simulink model "PI_controller"  (R2024b)
settings: Solver=FixedStepDiscrete  StartTime=0.0  StopTime=inf  FixedStep=0.02  RelTol=1e-3
undefined symbols (not defined in the file): brake, steering, throttle
libraries: ros2lib x5, slpidlib x1
settings Model: Creator=haavi  LastModifiedBy=haavi
settings OptimizationCC: DefaultParameterBehavior=Inlined  EnhancedBackFolding=on  PassReuseOutputArgsAs=Individual arguments  ZeroExternalMemoryAtStartup=off  ZeroInternalMemoryAtStartup=off  MaxStackSize=64  OptimizeBlockOrder=speed  DifferentSizesBufferReuse=on  EfficientTunableParamExpr=on
settings DebuggingCC: ParameterTunabilityLossMsg=error
settings SFSimCC: MATLABDynamicMemAlloc=off
settings RTWCC: Description=Embedded Coder  SystemTargetFile=ert.tlc  HardwareBoard=Robot Operating System 2 (ROS 2)  TLCOptions="-aInlineSetEventsForThisBaseRateFcn=TLC_FALSE -aSuppressMultiTaskScheduler=TLC_FALSE  -aRateBasedStepFcn=0"  TemplateMakefile=ert_default_tmf  Toolchain=Colcon Tools  TargetLang=C++
settings CodeAppCC: ForceParamTrailComments=on  IgnoreCustomStorageClasses=off  OperatorAnnotations=on  SimulinkDataObjDesc=on  SFDataObjDesc=on  InsertBlockDesc=on
settings ERTTargetCC: CodeInterfacePackaging=C++ class  SupportContinuousTime=on  RootIOFormat=Structure reference

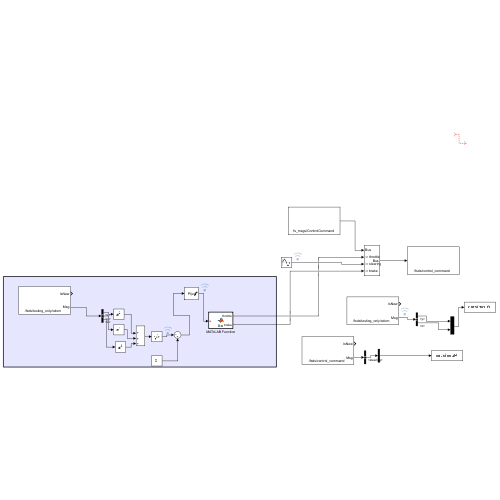
[thumbnail: Simulink's stored preview of the top-level diagram]
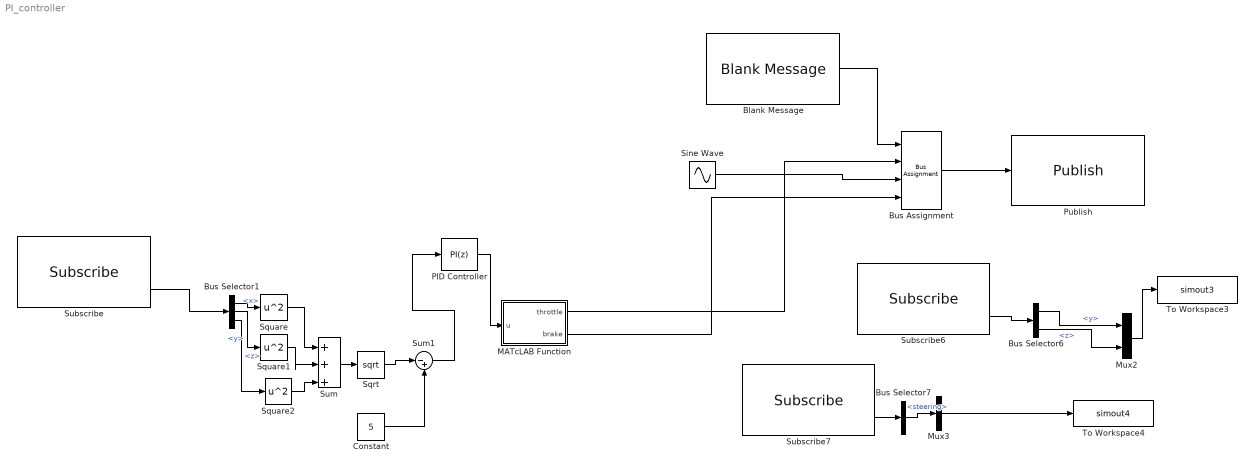
== system PI_controller ==
  Blank Message : ros2lib/Blank Message  messageClass=Message  entityType=fs_msgs/ControlCommand  messageType=fs_msgs/ControlCommand  SampleTime=0.02
  Bus Assignment : BusAssignment  AssignedSignals=throttle,steering,brake
  Bus Selector1 : BusSelector  OutputSignals=twist.twist.linear.x,twist.twist.linear.y,twist.twist.linear.z
  Bus Selector6 : BusSelector  OutputSignals=twist.twist.linear.y,twist.twist.angular.z
  Bus Selector7 : BusSelector  OutputSignals=steering
  Constant : Constant  Value=5
  MATcLAB Function : MATLAB Function  TreatAsAtomicUnit=on
  Mux2 : Mux  Inputs=2
  Mux3 : Mux  Inputs=1
  PID Controller : slpidlib/PID Controller  Controller=PI  Form=Parallel  TimeDomain=Discrete-time  UseExternalTs=off  SampleTime=0.02  IntegratorMethod=Forward Euler  FilterMethod=Forward Euler  ControllerParametersSource=internal  P=0.04  I=0.003  UseKiTs=off  D=0.0003  UseExternalDerivativeSource=off  N=100  UseFilter=off  TunerSelectOption=Transfer Function Based (PID Tuner App)  InitialConditionSource=internal  InitialConditionForIntegrator=0  InitialConditionForFilter=0  DifferentiatorICPrevScaledInput=0  ExternalReset=none  TrackingMode=off  Kt=1  LimitOutput=on  SatLimitsSource=internal  UpperSaturationLimit=1  LowerSaturationLimit=-1  LinearizeAsGain=off  AntiWindupMode=back-calculation  Kb=1  LimitIntegrator=off  UpperIntegratorSaturationLimit=0  LowerIntegratorSaturationLimit=1  POutMin=[]  POutMax=[]  IOutMin=[]  IOutMax=[]  DOutMin=[]  DOutMax=[]  NOutMin=[]  NOutMax=[]  SumOutMin=[]  SumOutMax=[]  SaturationOutMin=[]  SaturationOutMax=[]  PParamMin=[]  PParamMax=[]  IParamMin=[]  IParamMax=[]  DParamMin=[]  DParamMax=[]  NParamMin=[]  NParamMax=[]  KbParamMin=[]  KbParamMax=[]  KtParamMin=[]  KtParamMax=[]  KbOutMin=[]  KbOutMax=[]  KtOutMin=[]  KtOutMax=[]  IntegratorOutMin=[]  IntegratorOutMax=[]  FilterOutMin=[]  FilterOutMax=[]  SumI1OutMin=[]  SumI1OutMax=[]  SumI2OutMin=[]  SumI2OutMax=[]  SumI3OutMin=[]  SumI3OutMax=[]  SumI4OutMin=[]  SumI4OutMax=[]  SumDOutMin=[]  SumDOutMax=[]  DifferentiatorOutMin=[]  DifferentiatorOutMax=[]  FilterDiffOutCoefMin=[]  FilterDiffOutCoefMax=[]  ReciprocalOutMin=[]  ReciprocalOutMax=[]  SumDenOutMin=[]  SumDenOutMax=[]  SumNumOutMin=[]  SumNumOutMax=[]  DivideOutMin=[]  DivideOutMax=[]  UdiffTsProdOutMin=[]  UdiffTsProdOutMax=[]  NTsProdOutMin=[]  NTsProdOutMax=[]  UintegralTsProdOutMin=[]  UintegralTsProdOutMax=[]  UngainTsProdOutMin=[]  UngainTsProdOutMax=[]  ClampingZeroOutDataTypeStr=Inherit: Inherit via back propagation  ClampingZeroOutMin=[]  ClampingZeroOutMax=[]  FilterDenConstantOutDataTypeStr=Inherit: Inherit via back propagation  FilterDenConstantOutMin=[]  FilterDenConstantOutMax=[]  PCopyOutDataTypeStr=Inherit: Inherit via back propagation  PCopyOutMin=[]  PCopyOutMax=[]  NCopyOutDataTypeStr=Inherit: Inherit via back propagation  NCopyOutMin=[]  NCopyOutMax=[]  IntegratorContinuousStateAttributes=''  IntegratorStateMustResolveToSignalObject=off  IntegratorRTWStateStorageClass=Auto  FilterContinuousStateAttributes=''  FilterStateMustResolveToSignalObject=off  FilterRTWStateStorageClass=Auto  ParallelPVariant=InternalParameters  IdealPVariant=Disabled  IVariant=InternalParameters  DVariant=Disabled  IntegratorVariant=Discrete  SatVariant=Enabled  AWVariant=BackCalculation  PCopyVariant=Disabled  TRVariant=Disabled  FdbkBlocksVariant=Forward  IdealPFdbkVariant=Disabled  SatFdbkVariant=Disabled  DerivativeFilterVariant=Disabled  NVariant=Disabled  NCopyVariant=Disabled_SignalSpec  FilterICVariant=Disabled  IntegratorICVariant=InternalICs  ExternalResetVariant=Disabled  TRSumVariant=Passthrough  SumFdbkVariant=Disabled  SumVariant=Sum_PI  TsampFilterVariant=InternalTs  TsampNgainVariant=Passthrough  TsampIntegralVariant=Disabled_SignalSpec  ExternalSaturationOutDataTypeStr=Inherit: Same as second input  DerivativeSourceVariant=Disabled  PreIntVariant=InternalPreInt
  Publish : ros2lib/Publish  topicSource=Select from ROS network  topic=/fsds/control_command  messageType=fs_msgs/ControlCommand  QOSHistory=Keep last  QOSDepth=1  QOSReliability=Reliable  QOSDurability=Volatile  QOSDeadline=Inf  QOSLifespan=Inf  QOSLiveliness=Automatic  QOSLeaseDuration=Inf  QOSAvoidROSNamespaceConventions=off
  Sine Wave : Sin  Amplitude=0.01  Frequency=10  SampleTime=0
  Sqrt : Sqrt
  Square : Math  Operator=square
  Square1 : Math  Operator=square
  Square2 : Math  Operator=square
  Subscribe : ros2lib/Subscribe  topicSource=Select from ROS network  topic=/fsds/testing_only/odom  messageType=nav_msgs/Odometry  sampleTime=-1  QOSHistory=Keep all  QOSDepth=1  QOSReliability=Reliable  QOSDurability=Volatile  QOSDeadline=Inf  QOSLifespan=Inf  QOSLiveliness=Automatic  QOSLeaseDuration=Inf  QOSAvoidROSNamespaceConventions=off
  Subscribe6 : ros2lib/Subscribe  topicSource=Select from ROS network  topic=/fsds/testing_only/odom  messageType=nav_msgs/Odometry  sampleTime=0.02  QOSHistory=Keep last  QOSDepth=1  QOSReliability=Reliable  QOSDurability=Volatile  QOSDeadline=Inf  QOSLifespan=Inf  QOSLiveliness=Automatic  QOSLeaseDuration=Inf  QOSAvoidROSNamespaceConventions=off
  Subscribe7 : ros2lib/Subscribe  topicSource=Select from ROS network  topic=/fsds/control_command  messageType=fs_msgs/ControlCommand  sampleTime=0.02  QOSHistory=Keep last  QOSDepth=1  QOSReliability=Reliable  QOSDurability=Volatile  QOSDeadline=Inf  QOSLifespan=Inf  QOSLiveliness=Automatic  QOSLeaseDuration=Inf  QOSAvoidROSNamespaceConventions=off
  Sum : Sum  Inputs=|+++
  Sum1 : Sum  Inputs=|-+
  To Workspace3 : ToWorkspace  VariableName=simout3  SaveFormat=Timeseries  SampleTime=-1
  To Workspace4 : ToWorkspace  VariableName=simout4  SaveFormat=Timeseries  SampleTime=-1
  wires:
  Blank Message/1 -> Bus Assignment/1
  Bus Assignment/1 -> Publish/1
  ? -> ?
  Subscribe6/2 -> Bus Selector6/1
  Subscribe7/2 -> Bus Selector7/1
  Mux2/1 -> To Workspace3/1
  Mux3/1 -> To Workspace4/1
  Bus Selector6/1 -> Mux2/1  "<y>"
  Bus Selector7/1 -> Mux3/1  "<steering>"
  Sine Wave/1 -> Bus Assignment/3
  Bus Selector1/1 -> Square/1  "<x>"
  Sqrt/1 -> Sum1/1
  Bus Selector1/2 -> Square1/1  "<y>"
  PID Controller/1 -> MATcLAB Function/1(u)
  Sum1/1 -> PID Controller/1
  Square1/1 -> Sum/2
  Sum/1 -> Sqrt/1
  Constant/1 -> Sum1/2
  Bus Selector1/3 -> Square2/1  "<z>"
  Square/1 -> Sum/1
  Square2/1 -> Sum/3
  Subscribe/2 -> Bus Selector1/1
  MATcLAB Function/2(brake) -> Bus Assignment/4
  MATcLAB Function/1(throttle) -> Bus Assignment/2
  Bus Selector6/2 -> Mux2/2  "<z>"

== matlab function PI_controller/MATcLAB Function ==
  data: u input; throttle output; brake output
function [throttle, brake] = fcn(u)
       throttle = max(u, 0);
       brake = max(-u, 0);
   end
